simulink model "WaveStar"  (R2020b)
settings: Solver=ode4  StartTime=0  StopTime=141.2  FixedStep=0.001  MaxStep=0.001  RelTol=1e-3  EnableMultiTasking=on
values from neighbouring files (symbols this model uses):
  cc = 10.0    (= 10)    [controller_init.m]
  kc = 0    [controller_init.m]
  L_AB = 0.412    [controller_init.m]
  L_AC = 0.2    [controller_init.m]
  mc = 0    [controller_init.m]
  McSat = inf    [controller_init.m]
  simu = simulationClass()    [wecSimInputFile.m]
  xPcTs = 0.001    [controller_init.m]
undefined symbols (not defined in the file or in its folder): body, constraint, geometry, HPfreq, hydroData, LPfreq, pto, X, Y, Z
libraries: nesl_utility x36, sm_lib x26, WECSim_Lib_Body_Elements x5, simulink x2, WECSim_Lib_Constraints x2, WECSim_Lib_Frames x1
(part 1 of 2)
settings Model: Creator=kmruehl  LastModifiedBy=akeeste
settings SolverCC: ZeroCrossControl=DisableAll  AutoInsertRateTranBlk=on
settings DataIOCC: ReturnWorkspaceOutputs=off
settings OptimizationCC: LifeSpan=inf  SimCompilerOptimization=on
settings DebuggingCC: SFUnexpectedBacktrackingDiag=warning  SFNoUnconditionalDefaultTransitionDiag=warning  SFExecutionAtInitializationDiag=none  ArithmeticOperatorsInVariantConditions=warning
settings ModelReferenceCC: ModelReferenceMinAlgLoopOccurrences=on
settings SFSimCC: SimUseLocalCustomCode=off  CustomCodeUndefinedFunction=UseInterfaceOnly
settings RTWCC: RTWUseLocalCustomCode=off
settings CodeAppCC: StateflowObjectComments=on
settings GRTTargetCC: TargetLangStandard=C89/C90 (ANSI)
settings ConfigComp: CovMetricSettings=dw  CovSaveCumulativeToWorkspaceVar=on  CovSaveSingleToWorkspaceVar=on  CovExternalEMLEnable=off
settings SimscapeCC: SimscapeNormalizeSystem=off
settings ExplorerConfigSet: SimMechanicsOpenEditorOnUpdate=off  InternalSimMechanicsExplorerSettings="<ExplorerConfiguration><canonicalview>default</canonicalview><AnimationSetting><BasePlaybackSpeed>1.0</BasePlaybackSpeed><PlaybackSpeedFactor>1.0</PlaybackSpeedFactor></AnimationSetting><TilePanel><TileInfo><Tiles Columns=\"2\" Count=\"4\" Rows=\"2\"><Column Left=\"2\" Weight=\"0.4998\"/><Column Left=\"667\" Weight=\"0.5002\"/><Column Left=\"1333\"/><Row Top=\"2\" Weight=\"0.4997\"/><Row Top=\"952\" Weight=\"0.5003\"/><Row Top=\"1904\"/><Tile Height=\"1\" Width=\"1\" X=\"0\" Y=\"0\"/><Tile Height=\"1\" Width=\"1\" X=\"0\" Y=\"1\"/><Tile Height=\"1\" Width=\"1\" X=\"1\" Y=\"0\"/><Tile Height=\"1\" Width=\"1\" X=\"1\" Y=\"1\"/></Tiles></TileInfo><SceneInfo><SceneViewer><BGColor><R>0.60000002384185791</R><G>0.60000002384185791</G><B>0.60000002384185791</B></BGColor><Camera><DoPerspective>off</DoPerspective><Position><X>0.12470049519875293</X><Y>-7.8483064192972183</Y><Z>0.41049948909937695</Z></Position><Center><X>0.12470049519875293</X><Y>2.8810501090381635e-07</Y><Z>0.41049948909937695</Z></Center><Up><X>0</X><Y>-0</Y><Z>1</Z></Up><ViewLimDist>1</ViewLimDist><YLim>1.4359338132666335</YLim><XLim>1.0010335616396511</XLim></Camera></SceneViewer><SceneViewer><BGColor><R>0.60000002384185791</R><G>0.60000002384185791</G><B>0.60000002384185791</B></BGColor><Camera><DoPerspective>off</DoPerspective><Position><X>0.32732511337828807</X><Y>-0.082581165896399134</Y><Z>7.1171098135796953</Z></Position><Center><X>0.32732511337828807</X><Y>-0.082581165896399134</Y><Z>0.45174407037336595</Z></Center><Up><X>0</X><Y>1</Y><Z>-0</Z></Up><ViewLimDist>1</ViewLimDist><YLim>1.40160176353799</YLim><XLim>0.97502731376555829</XLim></Camera></SceneViewer><SceneViewer><BGColor><R>0.60000002384185791</R><G>0.60000002384185791</G><B>0.60000002384185791</B></BGColor><Camera><DoPerspective>off</DoPerspective><Position><X>7.848306419447999</X><Y>0.086028706913199554</Y><Z>0.42305679091343457</Z></Position><Center><X>-3.0318302890464111e-07</X><Y>0.086028706913199554</Y><Z>0.42305679091343457</Z></Center><Up><X>-0</X><Y>0</Y><Z>1</Z></Up><ViewLimDist>1</ViewLimDist><YLim>1.4671457032424258</YLim><XLim>1.0243514633690476</XLim></Camera></SceneViewer><SceneViewer><BGColor><R>0.60000002384185791</R><G>0.60000002384185791</G><B>0.60000002384185791</B></BGColor><Camera><DoPerspective>off</DoPerspective><Position><X>4.3109367218514292</X><Y>-3.7387044463777657</Y><Z>4.7725637716535374</Z></Position><Center><X>-0.21521500504762375</X><Y>0.78744728052128776</Y><Z>0.24641204475448614</Z></Center><Up><X>-0.40824829046386307</X><Y>0.40824829046386307</Y><Z>0.81649658092772615</Z></Up><ViewLimDist>1</ViewLimDist><YLim>1.979107791195027</YLim><XLim>1.3788693730807347</XLim></Camera></SceneViewer></SceneInfo></TilePanel><MechEditorPanel><Cameras/><GfxPanelCameraMap/><VideoCreator><PlaybackSpeedRatio>1.0</PlaybackSpeedRatio><FrameRate>30</FrameRate><VideoFormat>Motion JPEG AVI</VideoFormat><FrameSize>auto</FrameSize></VideoCreator></MechEditorPanel></ExplorerConfiguration>"

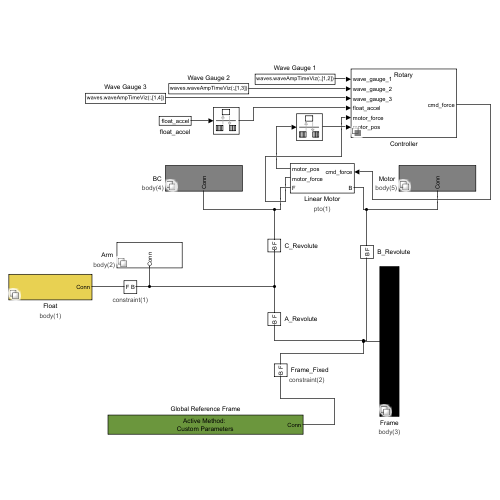
[thumbnail: Simulink's stored preview of the top-level diagram]
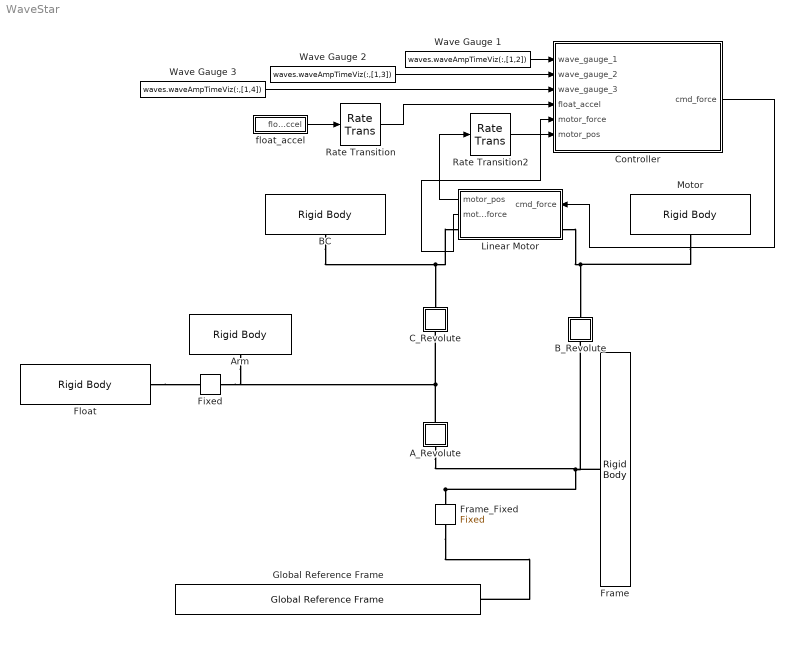
== system WaveStar ==
  A_Revolute : Subsystem
  Arm : WECSim_Lib_Body_Elements/Rigid Body  body=body(2)  h5File=hydroData/*.h5  geometryFile=geometry/*.stl  mass=0  inertia=0 0 0  inertiaProducts=0 0 0  nonHydro=0  nonlinearHydro=0  centerGravity=0 0 0  centerBuoyancy=0 0 0  dof=6  volume=0  displacement=0 0 0  axis=0 1 0  angle=0  option=0  cd=0 0 0  ca=0 0 0  area=0 0 0  VME=0  rgME=0 0 0  z=0 0 1
  BC : WECSim_Lib_Body_Elements/Rigid Body  body=body(4)  h5File=hydroData/*.h5  geometryFile=geometry/*.stl  mass=0  inertia=0 0 0  inertiaProducts=0 0 0  nonHydro=0  nonlinearHydro=0  centerGravity=0 0 0  centerBuoyancy=0 0 0  dof=6  volume=0  displacement=0 0 0  axis=0 1 0  angle=0  option=0  cd=0 0 0  ca=0 0 0  area=0 0 0  VME=0  rgME=0 0 0  z=0 0 1
  B_Revolute : Subsystem
  C_Revolute : Subsystem
  Controller : Subsystem  Variant=on  VariantControlMode=label  VariantControl=Variant1  LabelModeActiveChoice=VSS_Rotary
  Fixed : WECSim_Lib_Constraints/Fixed  constraint=constraint(1)  loc="0  0  0"  displacement=0 0 0  y=0 1 0  z=0 0 1  upperLimitSpecify=off  upperLimitBound=0  upperLimitTransitionRegionWidth=0  upperLimitStiffness=0  upperLimitDamping=0  lowerLimitSpecify=off  lowerLimitBound=0  lowerLimitTransitionRegionWidth=0  lowerLimitStiffness=0  lowerLimitDamping=0
      settings: AttributesFormatString=%<constraint>
  Float : WECSim_Lib_Body_Elements/Rigid Body  body=body(1)  h5File=hydroData/*.h5  geometryFile=geometry/*.stl  mass=0  inertia=0 0 0  inertiaProducts=0 0 0  nonHydro=0  nonlinearHydro=0  centerGravity=0 0 0  centerBuoyancy=0 0 0  dof=6  volume=0  displacement=0 0 0  axis=0 1 0  angle=0  option=0  cd=0 0 0  ca=0 0 0  area=0 0 0  VME=0  rgME=0 0 0  z=0 0 1
  Frame : WECSim_Lib_Body_Elements/Rigid Body  body=body(3)  h5File=hydroData/*.h5  geometryFile=geometry/*.stl  mass=0  inertia=0 0 0  inertiaProducts=0 0 0  nonHydro=0  nonlinearHydro=0  centerGravity=0 0 0  centerBuoyancy=0 0 0  dof=6  volume=0  displacement=0 0 0  axis=0 1 0  angle=0  option=0  cd=0 0 0  ca=0 0 0  area=0 0 0  VME=0  rgME=0 0 0  z=0 0 1
  Frame_Fixed : WECSim_Lib_Constraints/Fixed  constraint=constraint(2)  loc="0  0  0"  displacement=0 0 0  y=0 1 0  z=0 0 1  upperLimitSpecify=off  upperLimitBound=0  upperLimitTransitionRegionWidth=0  upperLimitStiffness=0  upperLimitDamping=0  lowerLimitSpecify=off  lowerLimitBound=0  lowerLimitTransitionRegionWidth=0  lowerLimitStiffness=0  lowerLimitDamping=0
      settings: AttributesFormatString=%<constraint>
  Global Reference Frame : WECSim_Lib_Frames/Global Reference Frame  waves=waves  simu=simu  InputMethod=Custom Parameters  InputFile=wecSimInputFile.m  mode=normal  explorer=off  solver=ode4  startTime=0  rampTime=100  endTime=400  dt=0.1  cicEndTime=60  stateSpace=0  WaveClass=regular  height=2.5  period=8  elevationFile=NOT DEFINED  spectrumFile=NOT DEFINED  direction=0  spread=1  spectrumType=NOT DEFINED  phaseSeed=0  option=EqualEnergy
  Linear Motor : Subsystem  mask(PTO){pto=pto(1)}
      mask prompts: pto "PTO Name:"
      mask help:
      | Constraints the follower to translational motion relative to the base, in
      | the PTO's Z-direction and adds PTO stiffness and damping. Also applies a
      | user-defined force and outputs extension, velocity, and acceleration.
      |
      |
      | The variable name input below must be 'pto(i)' where i=1,2,...
      | pto(i) must be defined in the input file with the following fields:
      |
      |     .name (required)
      |             String.
      |             PTO name. Must comply with Matlab's variable naming rules.
      |     .loc (optional)
      |             3x1 vector [x y z] in meters.
      |             PTO location. Default = [0 0 0]
      |     .k (optional)
      |             Float.
      |             PTO linear spring stiffness. Default = 0
      |     .c (optional)
      |             Float.
      |             PTO linear damping coefficient. Default = 0
      |     .orientation.z (optional)
      |             3x1 vector [x y z].
      |             Direction of the PTO's Z-coordinate. Default = [0 0 1]
      |     .orientation.y (optional)
      |             3x1 vector [x y z].
      |             Direction of the PTO's Y-coordinate. Default = [0 1 0]
      mask init:
      | if exist('pto','var')
      |     h=[gcb '/output'];
      |     responseName=['pto' num2str(pto.number) '_out'];
      |     set_param(h,'VariableName',responseName);
      | end
      | 
      | pto.checkLoc('W');
      settings: AttributesFormatString=%<pto>
      mask Help:
      | Constraints the follower to translational motion relative to the base, in
      | the PTO's Z-direction and adds PTO stiffness and damping. Also applies a
      | user-defined force and outputs extension, velocity, and acceleration.
      | 
      | 
      | The variable name input below must be 'pto(i)' where i=1,2,...
      | pto(i) must be defined in the input file with the following fields:
      | 
      |     .name (required)
      |             String.
      |             PTO name. Must comply with Matlab's variable naming rules.
      |     .loc (optional)
      |             3x1 vector [x y z] in meters.
      |             PTO location. Default = [0 0 0]
      |     .k (optional)
      |             Float.
      |             PTO linear spring stiffness. Default = 0
      |     .c (optional)
      |             Float.
      |             PTO linear damping coefficient. Default = 0
      |     .orientation.z (optional)
      |             3x1 vector [x y z].
      |             Direction of the PTO's Z-coordinate. Default = [0 0 1]
      |     .orientation.y (optional)
      |             3x1 vector [x y z].
      |             Direction of the PTO's Y-coordinate. Default = [0 1 0]
  Motor : WECSim_Lib_Body_Elements/Rigid Body  body=body(5)  h5File=hydroData/*.h5  geometryFile=geometry/*.stl  mass=0  inertia=0 0 0  inertiaProducts=0 0 0  nonHydro=0  nonlinearHydro=0  centerGravity=0 0 0  centerBuoyancy=0 0 0  dof=6  volume=0  displacement=0 0 0  axis=0 1 0  angle=0  option=0  cd=0 0 0  ca=0 0 0  area=0 0 0  VME=0  rgME=0 0 0  z=0 0 1
  Rate Transition : RateTransition  OutPortSampleTime=simu.dt
  Rate Transition2 : RateTransition  OutPortSampleTime=simu.dt
  Wave Gauge 1 : FromWorkspace  VariableName=waves.waveAmpTimeViz(:,[1,2])  SampleTime=simu.dt
  Wave Gauge 2 : FromWorkspace  VariableName=waves.waveAmpTimeViz(:,[1,3])  SampleTime=simu.dt
  Wave Gauge 3 : FromWorkspace  VariableName=waves.waveAmpTimeViz(:,[1,4])  SampleTime=simu.dt
  float_accel : Subsystem
  wires:
  Controller/1(cmd_force) -> Linear Motor/1(cmd_force)
  float_accel/1(float_accel) -> Rate Transition/1
  Linear Motor/1(motor_pos) -> Rate Transition2/1
  Linear Motor/2(motor_force) -> Controller/5(motor_force)
  Rate Transition2/1 -> Controller/6("motor_pos ")
  Rate Transition/1 -> Controller/4(float_accel)
  Wave Gauge 2/1 -> Controller/2(wave_gauge_2)
  Wave Gauge 1/1 -> Controller/1(wave_gauge_1)
  Wave Gauge 3/1 -> Controller/3(wave_gauge_3)
  connections:
  Frame_Fixed/RConn1 -- A_Revolute/LConn1 -- B_Revolute/LConn1 -- Frame/RConn1
  Frame_Fixed/LConn1 -- Global Reference Frame/RConn1
  Fixed/LConn1 -- Arm/RConn1 -- A_Revolute/RConn1 -- C_Revolute/LConn1
  BC/RConn1 -- C_Revolute/RConn1 -- Linear Motor/RConn1
  Motor/RConn1 -- Linear Motor/LConn1 -- B_Revolute/RConn1
  Float/RConn1 -- Fixed/RConn1

== system WaveStar/A_Revolute ==
  MATLAB Function : MATLAB Function  TreatAsAtomicUnit=on  mask{brkwy_trq=.25, brkwy_trq_unit=N*m, brkwy_vel=.1, brkwy_vel_unit=rad/s, Col_trq=.2, col_trq_unit=N*m, visc_coef=.001, visc_coef_unit=N*m/(rad/s)}
      mask prompts: brkwy_trq "Breakaway friction torque"; brkwy_vel "Breakaway friction velocity"; Col_trq "Coulomb friction torque"; visc_coef "Viscous friction coefficient"
  Ramp : simulink/Sources/Ramp  slope=1  start=0  InitialOutput=0
  Rate Transition1 : RateTransition  OutPortSampleTime=simu.dt
  Rotational PTO Actuation Torque1 : Subsystem  AncestorBlock=WECSim_Lib/PTOs/Rotational PTO Actuation Torque  mask(PTO){pto=pto(4)}
      mask prompts: pto "PTO Name:"
      mask help:
      | Constraints the follower to rotational motion relative to the base, about
      | the PTO's Y-direction and adds PTO stiffness and damping. Also applies a
      | user-defined torque and outputs extension, velocity and acceleration.
      |
      |
      | The variable name input below must be 'pto(i)' where i=1,2,...
      | pto(i) must be defined in the input file with the following fields:
      |
      |     .name (required)
      |             String.
      |             PTO name. Must comply with Matlab's variable naming rules.
      |     .loc (required)
      |             3x1 vector [x y z] in meters.
      |             PTO location. Default = [0 0 0]
      |     .k (optional)
      |             Float.
      |             PTO linear spring stiffness. Default = 0
      |     .c (optional)
      |             Float.
      |             PTO linear damping coefficient. Default = 0
      |     .orientation.z (optional)
      |             3x1 vector [x y z].
      |             Direction of the PTO's Z-coordinate. Default = [0 0 1]
      |     .orientation.y (optional)
      |             3x1 vector [x y z].
      |             Direction of the PTO's Y-coordinate. Default = [0 1 0]
      mask init:
      | if exist('pto','var')
      |     h=[gcb '/output'];
      |     responseName=['pto' num2str(pto.number) '_out'];
      |     set_param(h,'VariableName',responseName);
      | end
      | 
      | pto.checkLoc('E');
      settings: AttributesFormatString=%<pto>
      mask Help:
      | Constraints the follower to rotational motion relative to the base, about
      | the PTO's Y-direction and adds PTO stiffness and damping. Also applies a
      | user-defined torque and outputs extension, velocity and acceleration.
      | 
      | 
      | The variable name input below must be 'pto(i)' where i=1,2,...
      | pto(i) must be defined in the input file with the following fields:
      | 
      |     .name (required)
      |             String.
      |             PTO name. Must comply with Matlab's variable naming rules.
      |     .loc (required)
      |             3x1 vector [x y z] in meters.
      |             PTO location. Default = [0 0 0]
      |     .k (optional)
      |             Float.
      |             PTO linear spring stiffness. Default = 0
      |     .c (optional)
      |             Float.
      |             PTO linear damping coefficient. Default = 0
      |     .orientation.z (optional)
      |             3x1 vector [x y z].
      |             Direction of the PTO's Z-coordinate. Default = [0 0 1]
      |     .orientation.y (optional)
      |             3x1 vector [x y z].
      |             Direction of the PTO's Y-coordinate. Default = [0 1 0]
  F : PMIOPort  Side=Right
  B : PMIOPort  Port=2  Side=Left
  wires:
  Rotational PTO Actuation Torque1/1(Response) -> MATLAB Function/2(vel)
  MATLAB Function/1(t) -> Rotational PTO Actuation Torque1/1(Torque)
  Ramp/1 -> Rate Transition1/1
  Rate Transition1/1 -> MATLAB Function/1(time)
  connections:
  F/RConn1 -- Rotational PTO Actuation Torque1/RConn1
  B/RConn1 -- Rotational PTO Actuation Torque1/LConn1

== system WaveStar/B_Revolute ==
  MATLAB Function : MATLAB Function  TreatAsAtomicUnit=on  mask{brkwy_trq=.25, brkwy_trq_unit=N*m, brkwy_vel=.1, brkwy_vel_unit=rad/s, Col_trq=.2, col_trq_unit=N*m, visc_coef=.001, visc_coef_unit=N*m/(rad/s)}
      mask prompts: brkwy_trq "Breakaway friction torque"; brkwy_vel "Breakaway friction velocity"; Col_trq "Coulomb friction torque"; visc_coef "Viscous friction coefficient"
  Rotational PTO Actuation Torque1 : Subsystem  AncestorBlock=WECSim_Lib/PTOs/Rotational PTO Actuation Torque  mask(PTO){pto=pto(3)}
      mask prompts: pto "PTO Name:"
      mask help:
      | Constraints the follower to rotational motion relative to the base, about
      | the PTO's Y-direction and adds PTO stiffness and damping. Also applies a
      | user-defined torque and outputs extension, velocity and acceleration.
      |
      |
      | The variable name input below must be 'pto(i)' where i=1,2,...
      | pto(i) must be defined in the input file with the following fields:
      |
      |     .name (required)
      |             String.
      |             PTO name. Must comply with Matlab's variable naming rules.
      |     .loc (required)
      |             3x1 vector [x y z] in meters.
      |             PTO location. Default = [0 0 0]
      |     .k (optional)
      |             Float.
      |             PTO linear spring stiffness. Default = 0
      |     .c (optional)
      |             Float.
      |             PTO linear damping coefficient. Default = 0
      |     .orientation.z (optional)
      |             3x1 vector [x y z].
      |             Direction of the PTO's Z-coordinate. Default = [0 0 1]
      |     .orientation.y (optional)
      |             3x1 vector [x y z].
      |             Direction of the PTO's Y-coordinate. Default = [0 1 0]
      mask init:
      | if exist('pto','var')
      |     h=[gcb '/output'];
      |     responseName=['pto' num2str(pto.number) '_out'];
      |     set_param(h,'VariableName',responseName);
      | end
      | 
      | pto.checkLoc('E');
      settings: AttributesFormatString=%<pto>
      mask Help:
      | Constraints the follower to rotational motion relative to the base, about
      | the PTO's Y-direction and adds PTO stiffness and damping. Also applies a
      | user-defined torque and outputs extension, velocity and acceleration.
      | 
      | 
      | The variable name input below must be 'pto(i)' where i=1,2,...
      | pto(i) must be defined in the input file with the following fields:
      | 
      |     .name (required)
      |             String.
      |             PTO name. Must comply with Matlab's variable naming rules.
      |     .loc (required)
      |             3x1 vector [x y z] in meters.
      |             PTO location. Default = [0 0 0]
      |     .k (optional)
      |             Float.
      |             PTO linear spring stiffness. Default = 0
      |     .c (optional)
      |             Float.
      |             PTO linear damping coefficient. Default = 0
      |     .orientation.z (optional)
      |             3x1 vector [x y z].
      |             Direction of the PTO's Z-coordinate. Default = [0 0 1]
      |     .orientation.y (optional)
      |             3x1 vector [x y z].
      |             Direction of the PTO's Y-coordinate. Default = [0 1 0]
  F : PMIOPort  Side=Right
  B : PMIOPort  Port=2  Side=Left
  wires:
  Rotational PTO Actuation Torque1/1(Response) -> MATLAB Function/1(vel)
  MATLAB Function/1(t) -> Rotational PTO Actuation Torque1/1(Torque)
  connections:
  F/RConn1 -- Rotational PTO Actuation Torque1/RConn1
  B/RConn1 -- Rotational PTO Actuation Torque1/LConn1

== system WaveStar/C_Revolute ==
  MATLAB Function : MATLAB Function  TreatAsAtomicUnit=on  mask{brkwy_trq=.25, brkwy_trq_unit=N*m, brkwy_vel=.1, brkwy_vel_unit=rad/s, Col_trq=.2, col_trq_unit=N*m, visc_coef=.001, visc_coef_unit=N*m/(rad/s)}
      mask prompts: brkwy_trq "Breakaway friction torque"; brkwy_vel "Breakaway friction velocity"; Col_trq "Coulomb friction torque"; visc_coef "Viscous friction coefficient"
  Rotational PTO Actuation Torque1 : Subsystem  AncestorBlock=WECSim_Lib/PTOs/Rotational PTO Actuation Torque  mask(PTO){pto=pto(2)}
      mask prompts: pto "PTO Name:"
      mask help:
      | Constraints the follower to rotational motion relative to the base, about
      | the PTO's Y-direction and adds PTO stiffness and damping. Also applies a
      | user-defined torque and outputs extension, velocity and acceleration.
      |
      |
      | The variable name input below must be 'pto(i)' where i=1,2,...
      | pto(i) must be defined in the input file with the following fields:
      |
      |     .name (required)
      |             String.
      |             PTO name. Must comply with Matlab's variable naming rules.
      |     .loc (required)
      |             3x1 vector [x y z] in meters.
      |             PTO location. Default = [0 0 0]
      |     .k (optional)
      |             Float.
      |             PTO linear spring stiffness. Default = 0
      |     .c (optional)
      |             Float.
      |             PTO linear damping coefficient. Default = 0
      |     .orientation.z (optional)
      |             3x1 vector [x y z].
      |             Direction of the PTO's Z-coordinate. Default = [0 0 1]
      |     .orientation.y (optional)
      |             3x1 vector [x y z].
      |             Direction of the PTO's Y-coordinate. Default = [0 1 0]
      mask init:
      | if exist('pto','var')
      |     h=[gcb '/output'];
      |     responseName=['pto' num2str(pto.number) '_out'];
      |     set_param(h,'VariableName',responseName);
      | end
      | 
      | pto.checkLoc('E');
      settings: AttributesFormatString=%<pto>
      mask Help:
      | Constraints the follower to rotational motion relative to the base, about
      | the PTO's Y-direction and adds PTO stiffness and damping. Also applies a
      | user-defined torque and outputs extension, velocity and acceleration.
      | 
      | 
      | The variable name input below must be 'pto(i)' where i=1,2,...
      | pto(i) must be defined in the input file with the following fields:
      | 
      |     .name (required)
      |             String.
      |             PTO name. Must comply with Matlab's variable naming rules.
      |     .loc (required)
      |             3x1 vector [x y z] in meters.
      |             PTO location. Default = [0 0 0]
      |     .k (optional)
      |             Float.
      |             PTO linear spring stiffness. Default = 0
      |     .c (optional)
      |             Float.
      |             PTO linear damping coefficient. Default = 0
      |     .orientation.z (optional)
      |             3x1 vector [x y z].
      |             Direction of the PTO's Z-coordinate. Default = [0 0 1]
      |     .orientation.y (optional)
      |             3x1 vector [x y z].
      |             Direction of the PTO's Y-coordinate. Default = [0 1 0]
  F : PMIOPort  Side=Right
  B : PMIOPort  Port=2  Side=Left
  wires:
  Rotational PTO Actuation Torque1/1(Response) -> MATLAB Function/1(vel)
  MATLAB Function/1(t) -> Rotational PTO Actuation Torque1/1(Torque)
  connections:
  F/RConn1 -- Rotational PTO Actuation Torque1/RConn1
  B/RConn1 -- Rotational PTO Actuation Torque1/LConn1

== system WaveStar/Controller ==
  wave_gauge_1 : Inport
  wave_gauge_2 : Inport  Port=2
  wave_gauge_3 : Inport  Port=3
  float_accel : Inport  Port=4
  motor_force : Inport  Port=5
  "motor_pos " : Inport  Port=6
  Linear : Subsystem  VariantControl=VSS_Linear
  Rotary : Subsystem  VariantControl=VSS_Rotary
  cmd_force : Outport  VectorParamsAs1DForOutWhenUnconnected=off

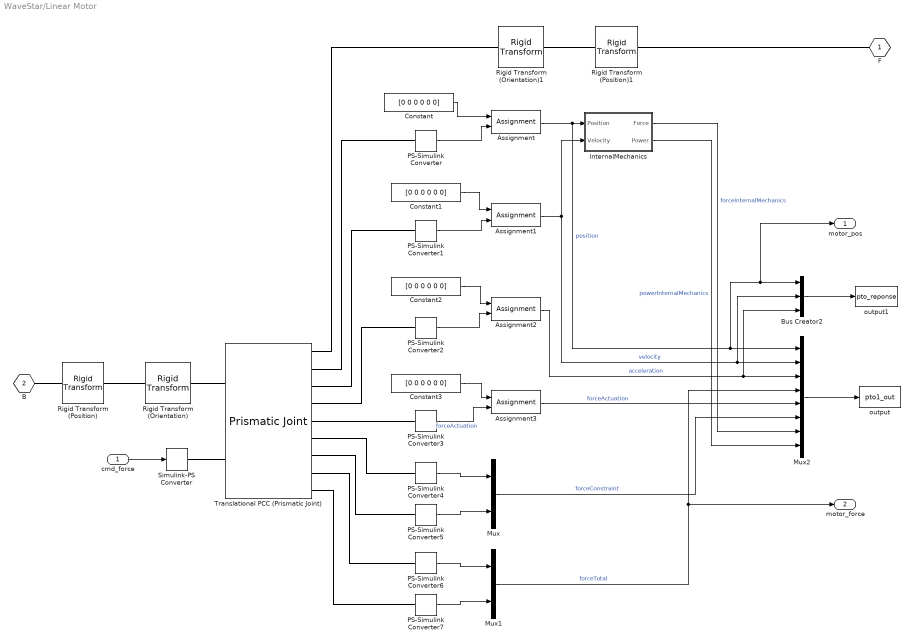
== system WaveStar/Linear Motor ==
  cmd_force : Inport
  Assignment{,1..3} (4 alike) : Assignment  IndexOptions=Index vector (dialog)  Indices=3  OutputSizes=1
  Bus Creator2 : BusCreator  Inputs=3
  Constant{,1..3} (4 alike) : Constant  Value=[0 0 0 0 0 0]
  InternalMechanics : Subsystem
  Mux : Mux  Inputs=2
  Mux1 : Mux  Inputs=2
  Mux2 : Mux  Inputs=8
  PS-Simulink Converter{,1..7} (8 alike) : nesl_utility/PS-Simulink Converter  PhysicalDomain=network_engine_domain  SubClassName=ps_output  LeftPortType=input  RightPortType=output  PseudoPeriodic=off  Frequencies=[]  VectorFormat=1-D array  Unit=1  AffineConversion=off
  Rigid Transform (Position) : sm_lib/Frames and Transforms/Rigid Transform  TranslationMethod=Cartesian  TranslationStandardOffset=0  TranslationStandardOffsetUnits=m  TranslationStandardAxis=+Z  TranslationCartesianOffset=pto.initial.displacement + pto.location  TranslationCartesianOffsetUnits=m  TranslationROffset=0  TranslationROffsetUnits=m  TranslationZOffset=0  TranslationZOffsetUnits=m  TranslationThetaOffset=0  TranslationThetaOffsetUnits=deg  RotationMethod=None  RotationAngleUnits=rad  RotationStandardAxis=+Y  RotationAngle=0  RotationArbitraryAxis=[0 1 0]  FollAlignAxisA=+X  BaseAlignAxisA=+Y  FollAlignAxisB=+Y  BaseAlignAxisB=+Z  RotationSequenceAxes=FollowerAxes  RotationSequence=XYX  RotationSequenceAngles=[0 0 0]  RotationSequenceAnglesUnits=deg  RotationMatrix=[1 0 0; 0 1 0; 0 0 1]  Quaternion=[1 0 0 0]
  Rigid Transform (Position)1 : sm_lib/Frames and Transforms/Rigid Transform  TranslationMethod=Cartesian  TranslationStandardOffset=0  TranslationStandardOffsetUnits=m  TranslationStandardAxis=+Z  TranslationCartesianOffset=pto.initial.displacement + pto.location  TranslationCartesianOffsetUnits=m  TranslationROffset=0  TranslationROffsetUnits=m  TranslationZOffset=0  TranslationZOffsetUnits=m  TranslationThetaOffset=0  TranslationThetaOffsetUnits=deg  RotationMethod=None  RotationAngleUnits=rad  RotationStandardAxis=+Y  RotationAngle=0  RotationArbitraryAxis=[0 1 0]  FollAlignAxisA=+X  BaseAlignAxisA=+Y  FollAlignAxisB=+Y  BaseAlignAxisB=+Z  RotationSequenceAxes=FollowerAxes  RotationSequence=XYX  RotationSequenceAngles=[0 0 0]  RotationSequenceAnglesUnits=deg  RotationMatrix=[1 0 0; 0 1 0; 0 0 1]  Quaternion=[1 0 0 0]
  Rigid Transform (Orientation) : sm_lib/Frames and Transforms/Rigid Transform  TranslationMethod=None  TranslationStandardOffset=0  TranslationStandardOffsetUnits=m  TranslationStandardAxis=+Z  TranslationCartesianOffset=0  TranslationCartesianOffsetUnits=m  TranslationROffset=0  TranslationROffsetUnits=m  TranslationZOffset=0  TranslationZOffsetUnits=m  TranslationThetaOffset=0  TranslationThetaOffsetUnits=deg  RotationMethod=RotationMatrix  RotationAngleUnits=rad  RotationStandardAxis=+Y  RotationAngle=0  RotationArbitraryAxis=[0 1 0]  FollAlignAxisA=+X  BaseAlignAxisA=+Y  FollAlignAxisB=+Y  BaseAlignAxisB=+Z  RotationSequenceAxes=FollowerAxes  RotationSequence=XYX  RotationSequenceAngles=[0 0 0]  RotationSequenceAnglesUnits=deg  RotationMatrix=pto.orientation.rotationMatrix  Quaternion=[1 0 0 0]
  Rigid Transform (Orientation)1 : sm_lib/Frames and Transforms/Rigid Transform  TranslationMethod=None  TranslationStandardOffset=0  TranslationStandardOffsetUnits=m  TranslationStandardAxis=+Z  TranslationCartesianOffset=0  TranslationCartesianOffsetUnits=m  TranslationROffset=0  TranslationROffsetUnits=m  TranslationZOffset=0  TranslationZOffsetUnits=m  TranslationThetaOffset=0  TranslationThetaOffsetUnits=deg  RotationMethod=RotationMatrix  RotationAngleUnits=rad  RotationStandardAxis=+Y  RotationAngle=0  RotationArbitraryAxis=[0 1 0]  FollAlignAxisA=+X  BaseAlignAxisA=+Y  FollAlignAxisB=+Y  BaseAlignAxisB=+Z  RotationSequenceAxes=FollowerAxes  RotationSequence=XYX  RotationSequenceAngles=[0 0 0]  RotationSequenceAnglesUnits=deg  RotationMatrix=pto.orientation.rotationMatrix  Quaternion=[1 0 0 0]
  Simulink-PS Converter : nesl_utility/Simulink-PS Converter  PhysicalDomain=network_engine_domain  SubClassName=ps_input  LeftPortType=input  RightPortType=output  PseudoPeriodic=off  Frequencies=[]  NoiseDistribution=none  NoiseParameters=[]  Unit=1  AffineConversion=off  FilteringAndDerivatives=zero  SimscapeFilterOrder=1  InputFilterTimeConstant=0.001  UdotUserProvided=1
  Translational PCC (Prismatic Joint) : sm_lib/Joints/Prismatic Joint  JointMode=Normal  SenseConstraintForce=on  SenseConstraintForceX=off  SenseConstraintForceY=off  SenseConstraintForceZ=off  SenseConstraintTorque=on  SenseConstraintTorqueX=off  SenseConstraintTorqueY=off  SenseConstraintTorqueZ=off  SenseTotalForce=on  SenseTotalForceX=off  SenseTotalForceY=off  SenseTotalForceZ=off  SenseTotalTorque=on  SenseTotalTorqueX=off  SenseTotalTorqueY=off  SenseTotalTorqueZ=off  CompositeWrenchDir=BaseOnFollower  CompositeWrenchFrame=BaseFrame  EquilibriumPosition=0  EquilibriumPositionUnits=m  SpringStiffness=pto.stiffness  SpringStiffnessUnits=N/m  DampingCoefficient=pto.damping  DampingCoefficientUnits=N/(m/s)  TorqueActuationMode=InputTorque  MotionActuationMode=ComputedMotion  SensePosition=on  SenseVelocity=on  SenseAcceleration=on  SenseTorqueForce=on  SenseLowerLimitTorqueForce=off  SenseUpperLimitTorqueForce=off  LowerLimitSpecify=off  LowerLimitBound=-1  LowerLimitBoundUnits=m  LowerLimitStiffness=1e6  LowerLimitStiffnessUnits=N/m  LowerLimitDamping=1e3  LowerLimitDampingUnits=N/(m/s)  LowerLimitTransitionRegionWidth=1e-4  LowerLimitTransitionRegionWidthUnits=m  UpperLimitSpecify=off  UpperLimitBound=1  UpperLimitBoundUnits=m  UpperLimitStiffness=1e6  UpperLimitStiffnessUnits=N/m  UpperLimitDamping=1e3  UpperLimitDampingUnits=N/(m/s)  UpperLimitTransitionRegionWidth=1e-4  UpperLimitTransitionRegionWidthUnits=m  PositionTargetSpecify=off  PositionTargetPriority=High  PositionTargetValue=0  PositionTargetValueUnits=m  VelocityTargetSpecify=off  VelocityTargetPriority=High  VelocityTargetValue=0  VelocityTargetValueUnits=m/s
  output : ToWorkspace  VariableName=pto1_out  SaveFormat=Structure With Time  SampleTime=-1
      settings: Decimation=round(simu.dtOut/simu.dt,0)
  output1 : ToWorkspace  VariableName=pto_reponse  SaveFormat=Structure With Time  SampleTime=-1
      settings: Decimation=round(simu.dtOut/simu.dt,0)
  F : PMIOPort  Side=Right
  B : PMIOPort  Port=2  Side=Left
  motor_pos : Outport  VectorParamsAs1DForOutWhenUnconnected=off
  motor_force : Outport  Port=2  VectorParamsAs1DForOutWhenUnconnected=off
  wires:
  Assignment/1 -> Mux2/1, motor_pos/1, Bus Creator2/1, InternalMechanics/1(Position)  "position"
  Assignment1/1 -> Mux2/2, Bus Creator2/2, InternalMechanics/2(Velocity)  "velocity"
  Assignment2/1 -> Mux2/3, Bus Creator2/3  "acceleration"
  cmd_force/1 -> Simulink-PS Converter/1
  Mux2/1 -> output/1
  Mux/1 -> Mux2/6  "forceConstraint"
  Mux1/1 -> motor_force/1, Mux2/4  "forceTotal"
  PS-Simulink Converter4/1 -> Mux/1
  PS-Simulink Converter5/1 -> Mux/2
  PS-Simulink Converter6/1 -> Mux1/1
  PS-Simulink Converter7/1 -> Mux1/2
  Assignment3/1 -> Mux2/5  "forceActuation"
  Constant/1 -> Assignment/1
  PS-Simulink Converter/1 -> Assignment/2
  Constant1/1 -> Assignment1/1
  PS-Simulink Converter1/1 -> Assignment1/2
  Constant2/1 -> Assignment2/1
  PS-Simulink Converter2/1 -> Assignment2/2
  InternalMechanics/1(Force) -> Mux2/7  "forceInternalMechanics"
  InternalMechanics/2(Power) -> Mux2/8  "powerInternalMechanics"
  Constant3/1 -> Assignment3/1
  PS-Simulink Converter3/1 -> Assignment3/2  "forceActuation"
  Bus Creator2/1 -> output1/1
  connections:
  Rigid Transform (Position)/RConn1 -- Rigid Transform (Orientation)/LConn1
  Rigid Transform (Position)1/RConn1 -- Rigid Transform (Orientation)1/LConn1
  Simulink-PS Converter/RConn1 -- Translational PCC (Prismatic Joint)/LConn2
  Rigid Transform (Orientation)/RConn1 -- Translational PCC (Prismatic Joint)/LConn1
  Rigid Transform (Position)/LConn1 -- B/RConn1
  Translational PCC (Prismatic Joint)/RConn5 -- PS-Simulink Converter3/LConn1
  Translational PCC (Prismatic Joint)/RConn9 -- PS-Simulink Converter7/LConn1
  Rigid Transform (Orientation)1/RConn1 -- Translational PCC (Prismatic Joint)/RConn1
  Translational PCC (Prismatic Joint)/RConn4 -- PS-Simulink Converter2/LConn1
  Translational PCC (Prismatic Joint)/RConn7 -- PS-Simulink Converter5/LConn1
  Translational PCC (Prismatic Joint)/RConn3 -- PS-Simulink Converter1/LConn1
  Rigid Transform (Position)1/LConn1 -- F/RConn1
  Translational PCC (Prismatic Joint)/RConn8 -- PS-Simulink Converter6/LConn1
  Translational PCC (Prismatic Joint)/RConn2 -- PS-Simulink Converter/LConn1
  Translational PCC (Prismatic Joint)/RConn6 -- PS-Simulink Converter4/LConn1

== system WaveStar/float_accel ==
  Delay : Delay  DelayLength=1  InitialCondition=0
  Radial Acceleration : Selector  InputPortWidth=6  IndexOptions=Index vector (dialog)  Indices=[5]  OutputSizes=1
  float_accel : Outport  VectorParamsAs1DForOutWhenUnconnected=off
  wires:
  [acc1] -> Radial Acceleration/1
  Radial Acceleration/1 -> Delay/1
  Delay/1 -> float_accel/1

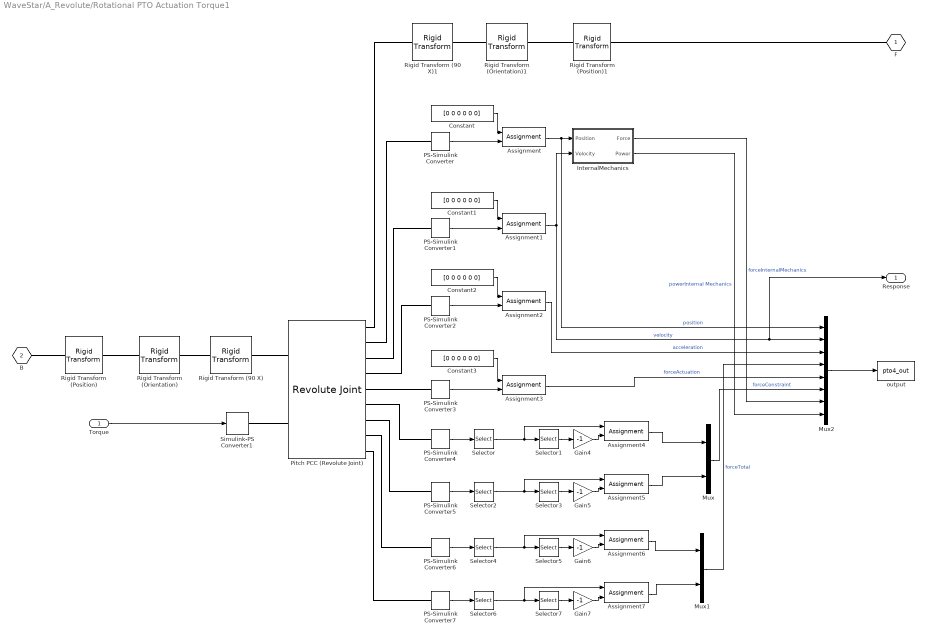
== system WaveStar/A_Revolute/Rotational PTO Actuation Torque1 ==
  Torque : Inport
  "Assignment " : Assignment  IndexOptions=Index vector (dialog)  Indices=5  OutputSizes=1
  Assignment1 : Assignment  IndexOptions=Index vector (dialog)  Indices=5  OutputSizes=1
  Assignment2 : Assignment  IndexOptions=Index vector (dialog)  Indices=5  OutputSizes=1
  Assignment3 : Assignment  IndexOptions=Index vector (dialog)  Indices=5  OutputSizes=1
  Assignment{4..7} (4 alike) : Assignment  DiagnosticForDimensions=Warning  IndexOptions=Index vector (dialog)  Indices=3  OutputSizes=1
  Constant{,1..3} (4 alike) : Constant  Value=[0 0 0 0 0 0]
  Gain{4..7} (4 alike) : Gain  Gain=-1
  InternalMechanics : Subsystem
  Mux : Mux  Inputs=2
  Mux1 : Mux  Inputs=2
  Mux2 : Mux  Inputs=8
  PS-Simulink Converter{,1..7} (8 alike) : nesl_utility/PS-Simulink Converter  PhysicalDomain=network_engine_domain  SubClassName=ps_output  LeftPortType=input  RightPortType=output  PseudoPeriodic=off  Frequencies=[]  VectorFormat=1-D array  Unit=1  AffineConversion=off
  Pitch PCC (Revolute Joint) : sm_lib/Joints/Revolute Joint  JointMode=Normal  SenseConstraintForce=on  SenseConstraintForceX=off  SenseConstraintForceY=off  SenseConstraintForceZ=off  SenseConstraintTorque=on  SenseConstraintTorqueX=off  SenseConstraintTorqueY=off  SenseConstraintTorqueZ=off  SenseTotalForce=on  SenseTotalForceX=off  SenseTotalForceY=off  SenseTotalForceZ=off  SenseTotalTorque=on  SenseTotalTorqueX=off  SenseTotalTorqueY=off  SenseTotalTorqueZ=off  CompositeWrenchDir=BaseOnFollower  CompositeWrenchFrame=BaseFrame  EquilibriumPosition=0  EquilibriumPositionUnits=deg  SpringStiffness=pto.stiffness  SpringStiffnessUnits=N*m/rad  DampingCoefficient=pto.damping  DampingCoefficientUnits=N*m/(rad/s)  TorqueActuationMode=InputTorque  MotionActuationMode=ComputedMotion  SensePosition=on  SenseVelocity=on  SenseAcceleration=on  SenseTorqueForce=on  SenseLowerLimitTorqueForce=off  SenseUpperLimitTorqueForce=off  LowerLimitSpecify=off  LowerLimitBound=-90  LowerLimitBoundUnits=deg  LowerLimitStiffness=1e4  LowerLimitStiffnessUnits=N*m/deg  LowerLimitDamping=10  LowerLimitDampingUnits=N*m/(deg/s)  LowerLimitTransitionRegionWidth=0.1  LowerLimitTransitionRegionWidthUnits=deg  UpperLimitSpecify=off  UpperLimitBound=90  UpperLimitBoundUnits=deg  UpperLimitStiffness=1e4  UpperLimitStiffnessUnits=N*m/deg  UpperLimitDamping=10  UpperLimitDampingUnits=N*m/(deg/s)  UpperLimitTransitionRegionWidth=0.1  UpperLimitTransitionRegionWidthUnits=deg  PositionTargetSpecify=off  PositionTargetPriority=High  PositionTargetValue=0  PositionTargetValueUnits=deg  VelocityTargetSpecify=off  VelocityTargetPriority=High  VelocityTargetValue=0  VelocityTargetValueUnits=deg/s
  Rigid Transform (Position) : sm_lib/Frames and Transforms/Rigid Transform  TranslationMethod=Cartesian  TranslationStandardOffset=0  TranslationStandardOffsetUnits=m  TranslationStandardAxis=+Z  TranslationCartesianOffset=pto.initial.displacement + pto.location  TranslationCartesianOffsetUnits=m  TranslationROffset=0  TranslationROffsetUnits=m  TranslationZOffset=0  TranslationZOffsetUnits=m  TranslationThetaOffset=0  TranslationThetaOffsetUnits=deg  RotationMethod=None  RotationAngleUnits=rad  RotationStandardAxis=+Y  RotationAngle=0  RotationArbitraryAxis=[0 1 0]  FollAlignAxisA=+X  BaseAlignAxisA=+Y  FollAlignAxisB=+Y  BaseAlignAxisB=+Z  RotationSequenceAxes=FollowerAxes  RotationSequence=XYX  RotationSequenceAngles=[0 0 0]  RotationSequenceAnglesUnits=deg  RotationMatrix=[1 0 0; 0 1 0; 0 0 1]  Quaternion=[1 0 0 0]
  Rigid Transform (Position)1 : sm_lib/Frames and Transforms/Rigid Transform  TranslationMethod=Cartesian  TranslationStandardOffset=0  TranslationStandardOffsetUnits=m  TranslationStandardAxis=+Z  TranslationCartesianOffset=pto.initial.displacement + pto.location  TranslationCartesianOffsetUnits=m  TranslationROffset=0  TranslationROffsetUnits=m  TranslationZOffset=0  TranslationZOffsetUnits=m  TranslationThetaOffset=0  TranslationThetaOffsetUnits=deg  RotationMethod=None  RotationAngleUnits=rad  RotationStandardAxis=+Y  RotationAngle=0  RotationArbitraryAxis=[0 1 0]  FollAlignAxisA=+X  BaseAlignAxisA=+Y  FollAlignAxisB=+Y  BaseAlignAxisB=+Z  RotationSequenceAxes=FollowerAxes  RotationSequence=XYX  RotationSequenceAngles=[0 0 0]  RotationSequenceAnglesUnits=deg  RotationMatrix=[1 0 0; 0 1 0; 0 0 1]  Quaternion=[1 0 0 0]
  Rigid Transform (90 X) : sm_lib/Frames and Transforms/Rigid Transform  TranslationMethod=None  TranslationStandardOffset=0  TranslationStandardOffsetUnits=m  TranslationStandardAxis=+Z  TranslationCartesianOffset=0  TranslationCartesianOffsetUnits=m  TranslationROffset=0  TranslationROffsetUnits=m  TranslationZOffset=0  TranslationZOffsetUnits=m  TranslationThetaOffset=0  TranslationThetaOffsetUnits=deg  RotationMethod=StandardAxis  RotationAngleUnits=deg  RotationStandardAxis=+X  RotationAngle=-90  RotationArbitraryAxis=[0 1 0]  FollAlignAxisA=+X  BaseAlignAxisA=+Y  FollAlignAxisB=+Y  BaseAlignAxisB=+Z  RotationSequenceAxes=FollowerAxes  RotationSequence=XYX  RotationSequenceAngles=[0 0 0]  RotationSequenceAnglesUnits=deg  RotationMatrix=[1 0 0; 0 1 0; 0 0 1]  Quaternion=[1 0 0 0]
  Rigid Transform (90 X)1 : sm_lib/Frames and Transforms/Rigid Transform  TranslationMethod=None  TranslationStandardOffset=0  TranslationStandardOffsetUnits=m  TranslationStandardAxis=+Z  TranslationCartesianOffset=0  TranslationCartesianOffsetUnits=m  TranslationROffset=0  TranslationROffsetUnits=m  TranslationZOffset=0  TranslationZOffsetUnits=m  TranslationThetaOffset=0  TranslationThetaOffsetUnits=deg  RotationMethod=StandardAxis  RotationAngleUnits=deg  RotationStandardAxis=+X  RotationAngle=-90  RotationArbitraryAxis=[0 1 0]  FollAlignAxisA=+X  BaseAlignAxisA=+Y  FollAlignAxisB=+Y  BaseAlignAxisB=+Z  RotationSequenceAxes=FollowerAxes  RotationSequence=XYX  RotationSequenceAngles=[0 0 0]  RotationSequenceAnglesUnits=deg  RotationMatrix=[1 0 0; 0 1 0; 0 0 1]  Quaternion=[1 0 0 0]
  Rigid Transform (Orientation) : sm_lib/Frames and Transforms/Rigid Transform  TranslationMethod=None  TranslationStandardOffset=0  TranslationStandardOffsetUnits=m  TranslationStandardAxis=+Z  TranslationCartesianOffset=0  TranslationCartesianOffsetUnits=m  TranslationROffset=0  TranslationROffsetUnits=m  TranslationZOffset=0  TranslationZOffsetUnits=m  TranslationThetaOffset=0  TranslationThetaOffsetUnits=deg  RotationMethod=RotationMatrix  RotationAngleUnits=rad  RotationStandardAxis=+Y  RotationAngle=0  RotationArbitraryAxis=[0 1 0]  FollAlignAxisA=+X  BaseAlignAxisA=+Y  FollAlignAxisB=+Y  BaseAlignAxisB=+Z  RotationSequenceAxes=FollowerAxes  RotationSequence=XYX  RotationSequenceAngles=[0 0 0]  RotationSequenceAnglesUnits=deg  RotationMatrix=pto.orientation.rotationMatrix  Quaternion=[1 0 0 0]
  Rigid Transform (Orientation)1 : sm_lib/Frames and Transforms/Rigid Transform  TranslationMethod=None  TranslationStandardOffset=0  TranslationStandardOffsetUnits=m  TranslationStandardAxis=+Z  TranslationCartesianOffset=0  TranslationCartesianOffsetUnits=m  TranslationROffset=0  TranslationROffsetUnits=m  TranslationZOffset=0  TranslationZOffsetUnits=m  TranslationThetaOffset=0  TranslationThetaOffsetUnits=deg  RotationMethod=RotationMatrix  RotationAngleUnits=rad  RotationStandardAxis=+Y  RotationAngle=0  RotationArbitraryAxis=[0 1 0]  FollAlignAxisA=+X  BaseAlignAxisA=+Y  FollAlignAxisB=+Y  BaseAlignAxisB=+Z  RotationSequenceAxes=FollowerAxes  RotationSequence=XYX  RotationSequenceAngles=[0 0 0]  RotationSequenceAnglesUnits=deg  RotationMatrix=pto.orientation.rotationMatrix  Quaternion=[1 0 0 0]
  Selector{,2,4,6} (4 alike) : Selector  InputPortWidth=3  IndexOptions=Index vector (dialog)  Indices=[1 3 2]  OutputSizes=1
  Selector{1,3,5,7} (4 alike) : Selector  InputPortWidth=3  IndexOptions=Index vector (dialog)  Indices=[3]  OutputSizes=1
  Simulink-PS Converter1 : nesl_utility/Simulink-PS Converter  PhysicalDomain=network_engine_domain  SubClassName=ps_input  LeftPortType=input  RightPortType=output  PseudoPeriodic=off  Frequencies=[]  NoiseDistribution=none  NoiseParameters=[]  Unit=1  AffineConversion=off  FilteringAndDerivatives=zero  SimscapeFilterOrder=1  InputFilterTimeConstant=0.001  UdotUserProvided=1
  output : ToWorkspace  VariableName=pto4_out  SaveFormat=Structure With Time  SampleTime=-1
      settings: Decimation=round(simu.dtOut/simu.dt,0)
  F : PMIOPort  Side=Right
  B : PMIOPort  Port=2  Side=Left
  Response : Outport  VectorParamsAs1DForOutWhenUnconnected=off
  wires:
  Torque/1 -> Simulink-PS Converter1/1
  "Assignment "/1 -> Mux2/1, InternalMechanics/1(Position)  "position"
  Assignment1/1 -> Response/1, Mux2/2, InternalMechanics/2(Velocity)  "velocity"
  Assignment2/1 -> Mux2/3  "acceleration"
  Selector2/1 -> Assignment5/1, Selector3/1
  Selector3/1 -> Gain5/1
  Gain5/1 -> Assignment5/2
  Selector/1 -> Assignment4/1, Selector1/1
  Selector1/1 -> Gain4/1
  Gain4/1 -> Assignment4/2
  Assignment5/1 -> Mux/2
  Assignment4/1 -> Mux/1
  Mux/1 -> Mux2/6  "forceConstraint"
  PS-Simulink Converter5/1 -> Selector2/1
  PS-Simulink Converter4/1 -> Selector/1
  Mux2/1 -> output/1
  Mux1/1 -> Mux2/4  "forceTotal"
  Selector6/1 -> Selector7/1, Assignment7/1
  Selector7/1 -> Gain7/1
  Gain7/1 -> Assignment7/2
  Selector4/1 -> Selector5/1, Assignment6/1
  Selector5/1 -> Gain6/1
  Gain6/1 -> Assignment6/2
  PS-Simulink Converter6/1 -> Selector4/1
  PS-Simulink Converter7/1 -> Selector6/1
  Assignment7/1 -> Mux1/2
  Assignment6/1 -> Mux1/1
  Constant/1 -> "Assignment "/1
  PS-Simulink Converter/1 -> "Assignment "/2
  Constant1/1 -> Assignment1/1
  PS-Simulink Converter1/1 -> Assignment1/2
  Constant2/1 -> Assignment2/1
  PS-Simulink Converter2/1 -> Assignment2/2
  Constant3/1 -> Assignment3/1
  PS-Simulink Converter3/1 -> Assignment3/2
  Assignment3/1 -> Mux2/5  "forceActuation"
  InternalMechanics/1(Force) -> Mux2/7  "forceInternalMechanics"
  InternalMechanics/2(Power) -> Mux2/8  "powerInternal Mechanics"
  connections:
  Rigid Transform (Position)1/LConn1 -- F/RConn1
  Rigid Transform (Position)/RConn1 -- Rigid Transform (Orientation)/LConn1
  Rigid Transform (Orientation)/RConn1 -- Rigid Transform (90 X)/LConn1
  Rigid Transform (Orientation)1/RConn1 -- Rigid Transform (90 X)1/LConn1
  Rigid Transform (Position)1/RConn1 -- Rigid Transform (Orientation)1/LConn1
  Rigid Transform (90 X)/RConn1 -- Pitch PCC (Revolute Joint)/LConn1
  Pitch PCC (Revolute Joint)/LConn2 -- Simulink-PS Converter1/RConn1
  Rigid Transform (Position)/LConn1 -- B/RConn1
  PS-Simulink Converter7/LConn1 -- Pitch PCC (Revolute Joint)/RConn9
  PS-Simulink Converter6/LConn1 -- Pitch PCC (Revolute Joint)/RConn8
  PS-Simulink Converter5/LConn1 -- Pitch PCC (Revolute Joint)/RConn7
  PS-Simulink Converter4/LConn1 -- Pitch PCC (Revolute Joint)/RConn6
  Pitch PCC (Revolute Joint)/RConn2 -- PS-Simulink Converter/LConn1
  Pitch PCC (Revolute Joint)/RConn3 -- PS-Simulink Converter1/LConn1
  PS-Simulink Converter2/LConn1 -- Pitch PCC (Revolute Joint)/RConn4
  PS-Simulink Converter3/LConn1 -- Pitch PCC (Revolute Joint)/RConn5
  Rigid Transform (90 X)1/RConn1 -- Pitch PCC (Revolute Joint)/RConn1
